simulink model "Avion_simulation_R2022b"  (R2022b)
settings: Solver=VariableStepAuto  StartTime=0.0  StopTime=100  RelTol=1e-3
undefined symbols (not defined in the file): A_lon, B_lon, C_lon, D_lon, Earth, ft, h_0, m, s, theta_0, V_0, WGS84
libraries: aerolibconvert2 x7, aerolibfltsims x2, simulink_extras x2, simulink x1, aerolibtransform2 x1, aerolibanimutils x1, aerolibanim x1
settings Model: Creator=georges  LastModifiedBy=georgesghazi
settings SolverCC: AlgebraicLoopSolver=TrustRegion
settings DataIOCC: ReturnWorkspaceOutputs=off
settings DebuggingCC: UnconnectedInputMsg=warning  UnconnectedOutputMsg=warning  UnconnectedLineMsg=warning  SFMachineParentedDataDiag=warning  ArithmeticOperatorsInVariantConditions=warning
settings ModelReferenceCC: EnableRefExpFcnMdlSchedulingChecks=on
settings SFSimCC: CustomCodeUndefinedFunction=UseInterfaceOnly

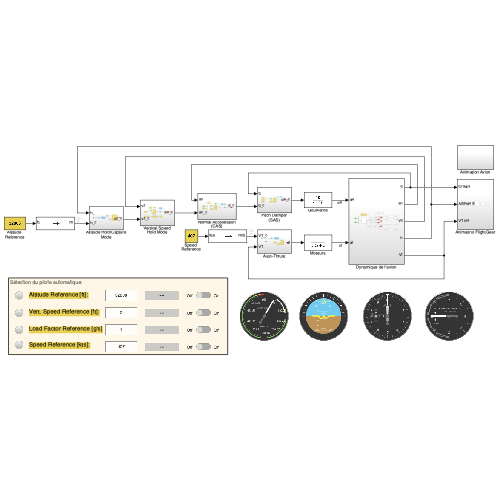
[thumbnail: Simulink's stored preview of the top-level diagram]
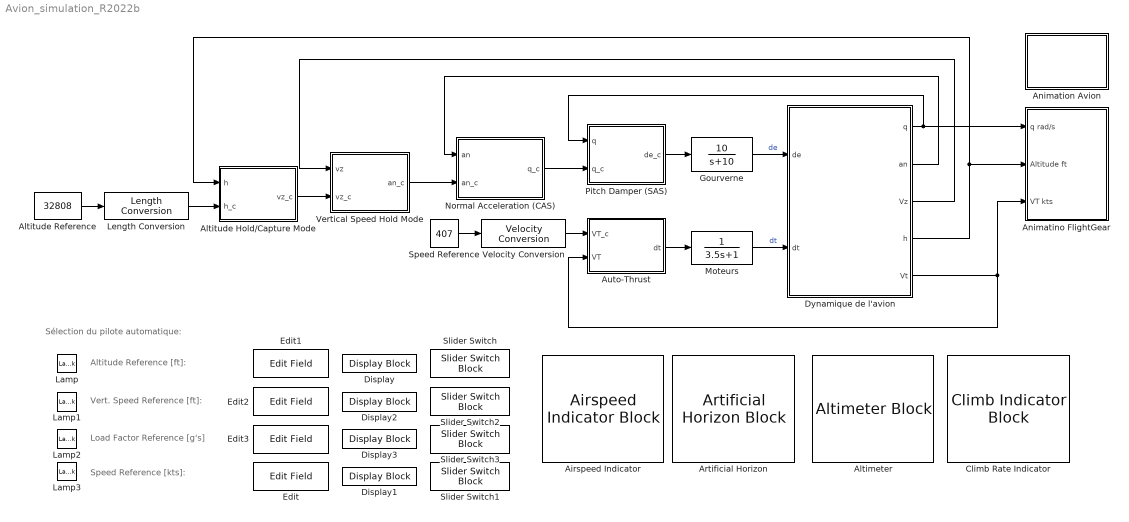
== system Avion_simulation_R2022b ==
  note: Altitude Reference [ft]:
  note: Sélection du pilote automatique:
  note: Speed Reference [kts]:
  note: Vert. Speed Reference [ft]:
  note: Load Factor Reference [g's]
  Airspeed Indicator : AirspeedIndicatorBlock  LabelPosition=Hide  ScaleMax=600
  Altimeter : AltimeterBlock  LabelPosition=Hide
  Altitude Reference : Constant  Value=32808
  Altitude Hold/Capture Mode : Subsystem
  Animatino FlightGear : Subsystem
  Animation Avion : Subsystem
  Artificial Horizon : ArtificialHorizonBlock  LabelPosition=Hide
  Auto-Thrust : Subsystem
  Climb Rate Indicator : ClimbIndicatorBlock  LabelPosition=Hide
  Display{,1..3} (4 alike) : DisplayBlock  LabelPosition=Hide  Format=long
  Dynamique de l'avion : Subsystem
  Edit{,1..3} (4 alike) : EditField  LabelPosition=Hide  ShowInitialText=on  Alignment=Center
  Gourverne : TransferFcn  Numerator=[10]  Denominator=[1 10]
  Lamp{,1..3} (4 alike) : LampBlock  LabelPosition=Hide
  Length Conversion : aerolibconvert2/Length Conversion  IU=ft  OU=m
  Moteurs : TransferFcn  Denominator=[3.5 1]
  Normal Acceleration (CAS) : Subsystem
  Pitch Damper (SAS) : Subsystem
  Slider Switch{,1..3} (4 alike) : SliderSwitchBlock  LabelPosition=Hide
      settings: Values={{'Off', 'On'}, [0 1]}
  Speed Reference : Constant  Value=407
  Velocity Conversion : aerolibconvert2/Velocity Conversion  IU=kts  OU=m/s
  Vertical Speed Hold Mode : Subsystem
  wires:
  Gourverne/1 -> Dynamique de l'avion/1(de)  "de"
  Moteurs/1 -> Dynamique de l'avion/2(dt)  "dt"
  Pitch Damper (SAS)/1(de_c) -> Gourverne/1
  Dynamique de l'avion/1(q) -> Animatino FlightGear/1(q rad/s), Pitch Damper (SAS)/1(q)
  Dynamique de l'avion/2(an) -> Normal Acceleration (CAS)/1(an)
  Auto-Thrust/1(dt) -> Moteurs/1
  Vertical Speed Hold Mode/1(an_c) -> Normal Acceleration (CAS)/2(an_c)
  Dynamique de l'avion/3(Vz) -> Vertical Speed Hold Mode/1(vz)
  Dynamique de l'avion/4(h) -> Altitude Hold/Capture Mode/1(h), Animatino FlightGear/2(Altitude ft)
  Altitude Reference/1 -> Length Conversion/1
  Speed Reference/1 -> Velocity Conversion/1
  Dynamique de l'avion/5(Vt) -> Animatino FlightGear/3(VT kts), Auto-Thrust/2(VT)
  Altitude Hold/Capture Mode/1(vz_c) -> Vertical Speed Hold Mode/2(vz_c)
  Normal Acceleration (CAS)/1(q_c) -> Pitch Damper (SAS)/2(q_c)
  Length Conversion/1 -> Altitude Hold/Capture Mode/2(h_c)
  Velocity Conversion/1 -> Auto-Thrust/1(VT_c)

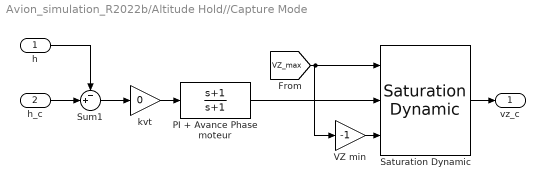
== system Avion_simulation_R2022b/Altitude Hold//Capture Mode ==
  h : Inport
  h_c : Inport  Port=2
  PI + Avance Phase moteur : TransferFcn  Numerator=[1 1]  Denominator=[1 1]
  Saturation Dynamic : simulink/Discontinuities/Saturation Dynamic  OutMin=[]  OutMax=[]  OutDataTypeStr=Inherit: Same as second input  OutDataType=fixdt(1, 16)  OutScaling=2^-10  DoSatur=off
  Sum1 : Sum  Inputs=-+|
  VZ min : Gain  Gain=-1
  kvt : Gain  Gain=0
  vz_c : Outport  VectorParamsAs1DForOutWhenUnconnected=off
  wires:
  Sum1/1 -> kvt/1
  h_c/1 -> Sum1/2
  kvt/1 -> PI + Avance Phase moteur/1
  PI + Avance Phase moteur/1 -> Saturation Dynamic/2
  h/1 -> Sum1/1
  Saturation Dynamic/1 -> vz_c/1
  [VZ_max] -> VZ min/1, Saturation Dynamic/1
  VZ min/1 -> Saturation Dynamic/3

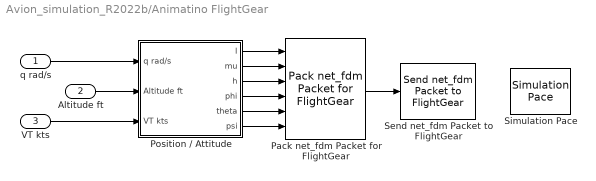
== system Avion_simulation_R2022b/Animatino FlightGear ==
  q rad/s : Inport
  Altitude ft : Inport  Port=2
  VT kts : Inport  Port=3
  Pack net_fdm Packet for FlightGear : aerolibfltsims/Pack net_fdm Packet for FlightGear  FlightGearVersion=v2019.1  ShowPositionAttitudeInputs=on  ShowVelocityAccelerationInputs=off  ShowControlSurfacePositionInputs=off  ShowEngineFuelInputs=off  ShowLandingGearInputs=off  ShowEnvironmentInputs=off  SampleTime=0.01  packetVersion=24
  Position / Attitude : Subsystem
  Send net_fdm Packet to FlightGear : aerolibfltsims/Send net_fdm Packet to FlightGear  DestinationIpAddress=127.0.0.1  DestinationPort=5502  LocalIpPort=-1  varLen=off  SampleTime=0.01
  Simulation Pace : aerolibanimutils/Simulation Pace  SimulationPace=1  SleepMode=MATLAB Thread  OutputPaceError=off  SampleTime=0.01
      settings: AttributesFormatString=%<SimulationPace> sec/sec
  wires:
  Altitude ft/1 -> Position / Attitude/2(Altitude ft)
  VT kts/1 -> Position / Attitude/3(VT kts)
  Position / Attitude/3(h) -> Pack net_fdm Packet for FlightGear/3
  Position / Attitude/5(theta) -> Pack net_fdm Packet for FlightGear/5
  q rad/s/1 -> Position / Attitude/1(q rad/s)
  Pack net_fdm Packet for FlightGear/1 -> Send net_fdm Packet to FlightGear/1
  Position / Attitude/2(mu) -> Pack net_fdm Packet for FlightGear/2
  Position / Attitude/6(psi) -> Pack net_fdm Packet for FlightGear/6
  Position / Attitude/1(I) -> Pack net_fdm Packet for FlightGear/1
  Position / Attitude/4(phi) -> Pack net_fdm Packet for FlightGear/4

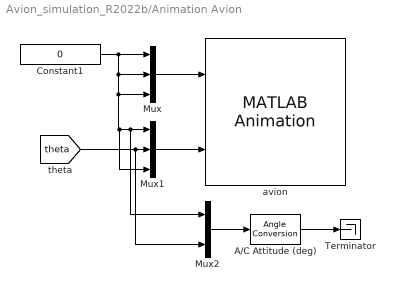
== system Avion_simulation_R2022b/Animation Avion ==
  A/C Attitude (deg) : aerolibconvert2/Angle Conversion  IU=rad  OU=deg
  Constant1 : Constant  Value=0
  Mux : Mux  Inputs=3
  Mux1 : Mux  Inputs=3
  Mux2 : Mux  Inputs=2
  Terminator : Terminator
  avion : aerolibanim/MATLAB Animation  Vehicles=1  Geometries='avion.ac'  BoundingBoxCoordinates=[-50,50,-50,50,-50,50]  CameraOffset=[250,-200,-10]  CameraViewAngle=4  SampleTime=0.1  FigurePosition=[865,477,405,248]
  wires:
  Mux/1 -> avion/1
  Constant1/1 -> Mux/2, Mux/3, Mux1/3, Mux2/1, Mux1/1, Mux/1
  [theta] -> Mux2/2, Mux1/2
  Mux1/1 -> avion/2
  Mux2/1 -> A/C Attitude (deg)/1
  A/C Attitude (deg)/1 -> Terminator/1

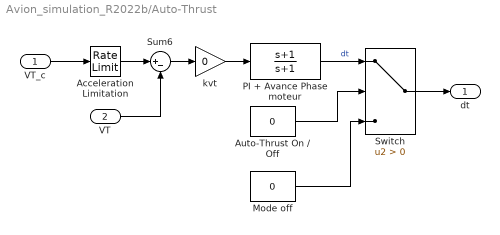
== system Avion_simulation_R2022b/Auto-Thrust ==
  VT_c : Inport
  VT : Inport  Port=2
  Acceleration Limitation : RateLimiter  RisingSlewLimit=0.01  FallingSlewLimit=-0.01  SampleTimeMode=inherited
  Auto-Thrust On / Off : Constant  Value=0
  Mode off : Constant  Value=0
  PI + Avance Phase moteur : TransferFcn  Numerator=[1 1]  Denominator=[1 1]
  Sum6 : Sum  Inputs=|+-
  Switch : Switch  Criteria=u2 > Threshold  SaturateOnIntegerOverflow=off  InputSameDT=off
  kvt : Gain  Gain=0
  dt : Outport  VectorParamsAs1DForOutWhenUnconnected=off
  wires:
  Sum6/1 -> kvt/1
  kvt/1 -> PI + Avance Phase moteur/1
  VT/1 -> Sum6/2
  VT_c/1 -> Acceleration Limitation/1
  Acceleration Limitation/1 -> Sum6/1
  Auto-Thrust On / Off/1 -> Switch/2
  PI + Avance Phase moteur/1 -> Switch/1  "dt"
  Mode off/1 -> Switch/3
  Switch/1 -> dt/1

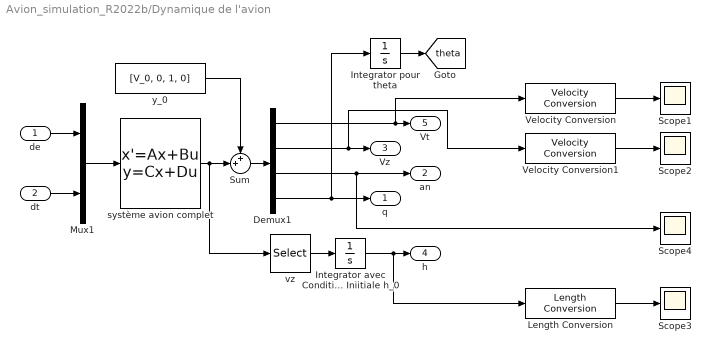
== system Avion_simulation_R2022b/Dynamique de l'avion ==
  de : Inport
  dt : Inport  Port=2
  Demux1 : Demux
  Integrator avec Condition Iniitiale h_0 : Integrator  InitialCondition=h_0
  Integrator pour theta : Integrator  InitialCondition=theta_0
  Length Conversion : aerolibconvert2/Length Conversion  IU=m  OU=ft
  Mux1 : Mux  Inputs=2
  Scope{1..4} (4 alike) : Scope
  Sum : Sum  Inputs=++|
  Velocity Conversion : aerolibconvert2/Velocity Conversion  IU=m/s  OU=kts
  Velocity Conversion1 : aerolibconvert2/Velocity Conversion  IU=m/s  OU=ft/min
  système avion complet : StateSpace  A=A_lon  B=B_lon  C=C_lon  D=D_lon  InitialCondition=0
  vz : Selector  InputPortWidth=4  IndexOptions=Index vector (dialog)  Indices=2  OutputSizes=1
  y_0 : Constant  Value=[V_0, 0, 1, 0]
  q : Outport  VectorParamsAs1DForOutWhenUnconnected=off
  an : Outport  Port=2  VectorParamsAs1DForOutWhenUnconnected=off
  Vz : Outport  Port=3  VectorParamsAs1DForOutWhenUnconnected=off
  h : Outport  Port=4  VectorParamsAs1DForOutWhenUnconnected=off
  Vt : Outport  Port=5  VectorParamsAs1DForOutWhenUnconnected=off
  tag scope: theta=global
  wires:
  Demux1/2 -> Velocity Conversion1/1, Vz/1
  Demux1/3 -> an/1, Scope4/1
  dt/1 -> Mux1/2
  de/1 -> Mux1/1
  Demux1/4 -> Integrator pour theta/1, q/1
  Demux1/1 -> Velocity Conversion/1, Vt/1
  vz/1 -> Integrator avec Condition Iniitiale h_0/1
  Integrator pour theta/1 -> [theta]
  système avion complet/1 -> vz/1, Sum/2
  Sum/1 -> Demux1/1
  y_0/1 -> Sum/1
  Mux1/1 -> système avion complet/1
  Velocity Conversion/1 -> Scope1/1
  Velocity Conversion1/1 -> Scope2/1
  Length Conversion/1 -> Scope3/1
  Integrator avec Condition Iniitiale h_0/1 -> Length Conversion/1, h/1

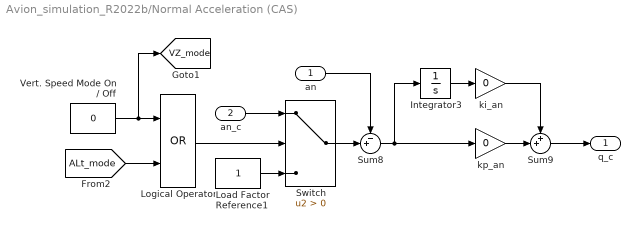
== system Avion_simulation_R2022b/Normal Acceleration (CAS) ==
  an : Inport
  an_c : Inport  Port=2
  Integrator3 : Integrator
  Load Factor Reference1 : Constant
  Logical Operator : Logic  Operator=OR  AllPortsSameDT=off  OutDataTypeStr=boolean
  Sum8 : Sum  Inputs=-+|
  Sum9 : Sum  Inputs=++|
  Switch : Switch  Criteria=u2 > Threshold  SaturateOnIntegerOverflow=off  InputSameDT=off
  Vert. Speed Mode On / Off : Constant  Value=0
  ki_an : Gain  Gain=0
  kp_an : Gain  Gain=0
  q_c : Outport  VectorParamsAs1DForOutWhenUnconnected=off
  tag scope: VZ_mode=global
  wires:
  kp_an/1 -> Sum9/2
  Integrator3/1 -> ki_an/1
  an/1 -> Sum8/1
  ki_an/1 -> Sum9/1
  Sum8/1 -> kp_an/1, Integrator3/1
  Sum9/1 -> q_c/1
  Switch/1 -> Sum8/2
  an_c/1 -> Switch/1
  [ALt_mode] -> Logical Operator/2
  Vert. Speed Mode On / Off/1 -> [VZ_mode], Logical Operator/1
  Logical Operator/1 -> Switch/2
  Load Factor Reference1/1 -> Switch/3

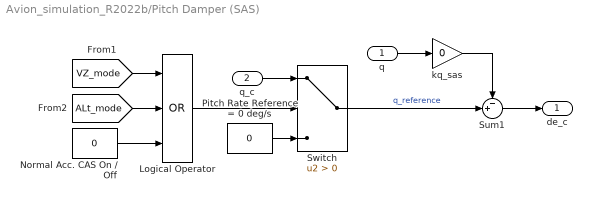
== system Avion_simulation_R2022b/Pitch Damper (SAS) ==
  q : Inport
  q_c : Inport  Port=2
  Logical Operator : Logic  Operator=OR  Inputs=3  AllPortsSameDT=off  OutDataTypeStr=boolean
  Normal Acc. CAS On / Off : Constant  Value=0
  Pitch Rate Reference = 0 deg/s : Constant  Value=0
  Sum1 : Sum  Inputs=-+|
  Switch : Switch  Criteria=u2 > Threshold  SaturateOnIntegerOverflow=off  InputSameDT=off
  kq_sas : Gain  Gain=0
  de_c : Outport  VectorParamsAs1DForOutWhenUnconnected=off
  wires:
  Sum1/1 -> de_c/1
  kq_sas/1 -> Sum1/1
  q/1 -> kq_sas/1
  Pitch Rate Reference = 0 deg/s/1 -> Switch/3
  [VZ_mode] -> Logical Operator/1
  [ALt_mode] -> Logical Operator/2
  Logical Operator/1 -> Switch/2
  q_c/1 -> Switch/1
  Normal Acc. CAS On / Off/1 -> Logical Operator/3
  Switch/1 -> Sum1/2  "q_reference"

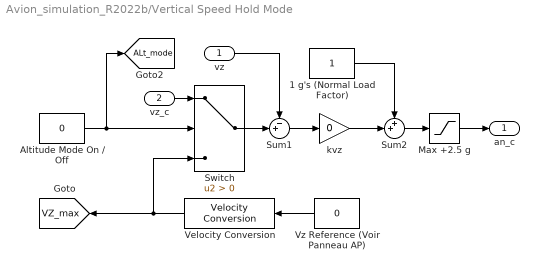
== system Avion_simulation_R2022b/Vertical Speed Hold Mode ==
  vz : Inport
  vz_c : Inport  Port=2
  1 g's (Normal Load Factor) : Constant
  Altitude Mode On / Off : Constant  Value=0
  Max +2.5 g : Saturate  UpperLimit=+2.5  LowerLimit=-1
  Sum1 : Sum  Inputs=-+|
  Sum2 : Sum  Inputs=++|
  Switch : Switch  Criteria=u2 > Threshold  SaturateOnIntegerOverflow=off  InputSameDT=off
  Velocity Conversion : aerolibconvert2/Velocity Conversion  IU=ft/min  OU=m/s
  Vz Reference (Voir Panneau AP) : Constant  Value=0
  kvz : Gain  Gain=0
  an_c : Outport  VectorParamsAs1DForOutWhenUnconnected=off
  tag scope: ALt_mode=global, VZ_max=global
  wires:
  vz/1 -> Sum1/1
  Sum1/1 -> kvz/1
  Max +2.5 g/1 -> an_c/1
  Sum2/1 -> Max +2.5 g/1
  kvz/1 -> Sum2/2
  1 g's (Normal Load Factor)/1 -> Sum2/1
  Vz Reference (Voir Panneau AP)/1 -> Velocity Conversion/1
  Switch/1 -> Sum1/2
  vz_c/1 -> Switch/1
  Velocity Conversion/1 -> Switch/3, [VZ_max]
  Altitude Mode On / Off/1 -> [ALt_mode], Switch/2

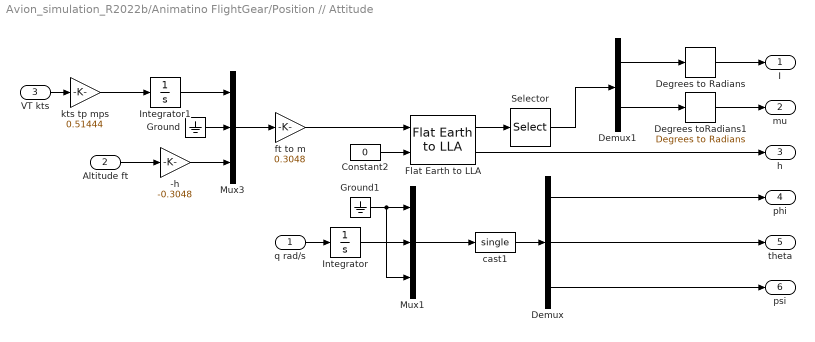
== system Avion_simulation_R2022b/Animatino FlightGear/Position // Attitude ==
  q rad/s : Inport
  Altitude ft : Inport  Port=2
  VT kts : Inport  Port=3
  -h : Gain  Gain=-0.3048
  Constant2 : Constant  Value=0
  Degrees to Radians : simulink_extras/Transformations/Degrees to Radians
  Degrees toRadians1 : simulink_extras/Transformations/Degrees to Radians
  Demux : Demux  Outputs=3
  Demux1 : Demux  Outputs=2
  Flat Earth to LLA : aerolibtransform2/Flat Earth to LLA  units=Metric (MKS)  ptype=Earth (WGS84)  F=1/298.257223563  R=6378137  refPosPort=off  LL0=[37.6637 -122.4778]  psi=0
  Ground : Ground
  Ground1 : Ground
  Integrator : Integrator
  Integrator1 : Integrator
  Mux1 : Mux  Inputs=3
  Mux3 : Mux  Inputs=3
  Selector : Selector  InputPortWidth=2  IndexOptions=Index vector (dialog)  Indices=[2 1]  OutputSizes=1
  cast1 : DataTypeConversion  OutDataTypeStr=single  RndMeth=Floor
  ft to m : Gain  Gain=0.3048
  kts tp mps : Gain  Gain=0.51444
  I : Outport
  mu : Outport  Port=2
  h : Outport  Port=3
  phi : Outport  Port=4
  theta : Outport  Port=5
  psi : Outport  Port=6
  wires:
  cast1/1 -> Demux/1
  Selector/1 -> Demux1/1
  Demux1/2 -> Degrees toRadians1/1
  Demux1/1 -> Degrees to Radians/1
  Demux/3 -> psi/1
  Demux/2 -> theta/1
  Demux/1 -> phi/1
  Ground/1 -> Mux3/2
  Altitude ft/1 -> -h/1
  Mux3/1 -> ft to m/1
  Flat Earth to LLA/1 -> Selector/1
  Flat Earth to LLA/2 -> h/1
  Constant2/1 -> Flat Earth to LLA/2
  Degrees to Radians/1 -> I/1
  Degrees toRadians1/1 -> mu/1
  ft to m/1 -> Flat Earth to LLA/1
  -h/1 -> Mux3/3
  q rad/s/1 -> Integrator/1
  VT kts/1 -> kts tp mps/1
  Integrator1/1 -> Mux3/1
  kts tp mps/1 -> Integrator1/1
  Mux1/1 -> cast1/1
  Integrator/1 -> Mux1/2
  Ground1/1 -> Mux1/3, Mux1/1
